simulink subsystem "Autonomous_sub"  (R2023b)
settings: Solver=VariableStepAuto  StartTime=0.0  StopTime=10.0  RelTol=1e-3
undefined symbols (not defined in the file): Auto_Deploy_Intake_Time, Auto_Deploy_Intake_Time2, Auto_Intake_Arm_Cycle_Delay_Time, Auto_Path_01, Auto_Path_02, Auto_Path_03, Auto_Path_04, Auto_Path_05, Auto_Path_06, Auto_Path_07, Auto_Path_08, Auto_Path_09, Auto_Path_10, Auto_Path_11, Auto_Path_12, Auto_Path_13, Auto_Path_Chooser, Auto_Shoot_Time, t_sample
libraries: simulink x11
settings Model: Creator=ander  LastModifiedBy=ander

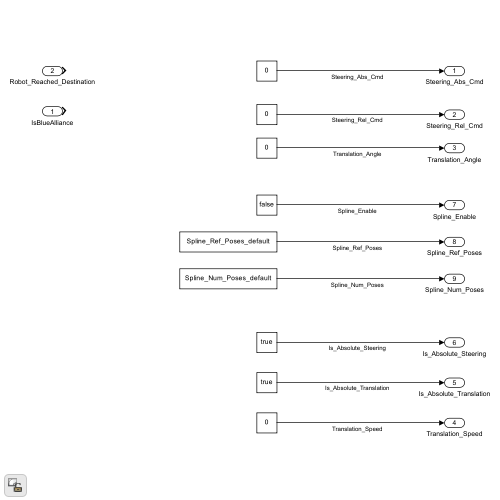
[thumbnail: Simulink's stored preview of the top-level diagram]
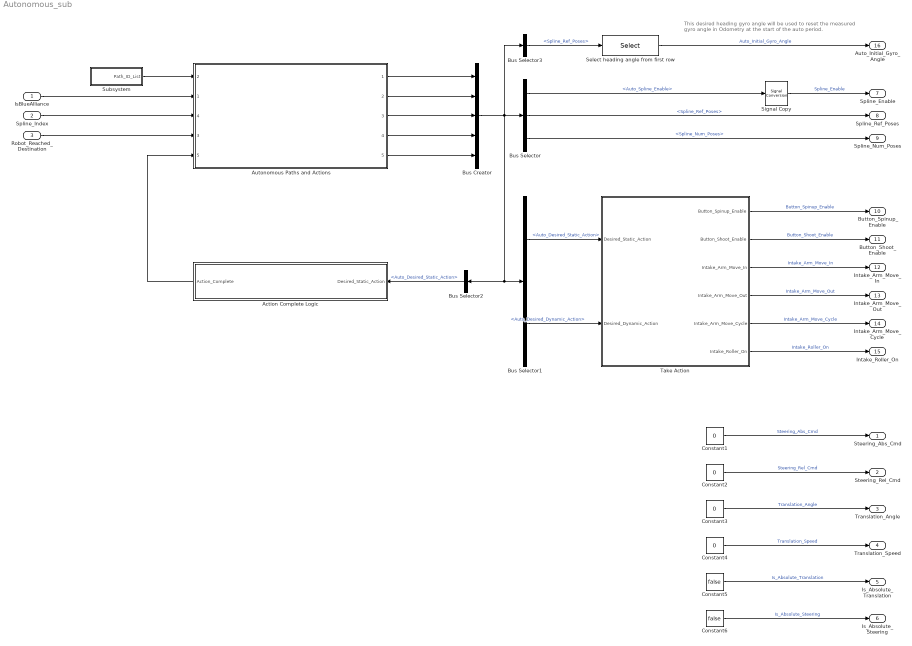
== system Autonomous_sub ==
  note: This desired heading gyro angle will be used to reset the measured gyro angle in Odometry at the start of the auto period.
  IsBlueAlliance : Inport
  Spline_Index : Inport  Port=2
  Robot_Reached_Destination : Inport  Port=3
  Action Complete Logic : Subsystem
  Autonomous Paths and Actions : Subsystem  ReferencedSubsystem=Autonomous_Paths_and_Actions_sub
      settings: PortSchema="{\"entries\":[{\"content\":{\"sides\":[{\"content\":{\"connectorIds\":[\"In2\",\"In1\",\"In4\",\"In3\",\"In5\"]},\"type\":\"ConnectorPlacement.EquallySpacedRectSide\",\"uuid\":\"294b2687-843c-4c6b-bb7a-4ddaa154855b\"},{\"content\":{\"connectorIds\":[\"Out1\",\"Out2\",\"Out3\",\"Out4\",\"Out5\"],\"side\":\"RIGHT\"},\"type\":\"ConnectorPlacement.EquallySpacedRectSide\",\"uuid\":\"d2e82f95-38dc-427a-93e1-a9041617c293\"},{\"content\":{\"side\":\"TOP\"},\"type\":\"ConnectorPlacement.EquallySpacedRectSide\",\"uuid\":\"31522bff-3666-4a04-81e4-ecf410bf1187\"}]},\"type\":\"ConnectorPlacement.EquallySpacedConnector\",\"uuid\":\"964fa79a-4b4c-4d0b-bc10-97a47e67b0ba\"}],\"packageUris\":[\"http://schema.mathworks.com/mf0/Connector/R2020b\"],\"version\":\"1.0\"}"
  Bus Creator : BusCreator  Inputs=5
  Bus Selector : BusSelector  OutputSignals=Auto_Spline_Enable,Spline_Ref_Poses,Spline_Num_Poses
  Bus Selector1 : BusSelector  OutputSignals=Auto_Desired_Static_Action,Auto_Desired_Dynamic_Action
  Bus Selector2 : BusSelector  OutputSignals=Auto_Desired_Static_Action
  Bus Selector3 : BusSelector  OutputSignals=Spline_Ref_Poses
  Constant{1..4} (4 alike) : Constant  Value=0
  Constant5 : Constant  Value=false
  Constant6 : Constant  Value=false
  Select heading angle from first row : Selector  NumberOfDimensions=2  InputPortWidth=3  IndexOptions=Index vector (dialog),Index vector (dialog)  Indices=[1],[4]  OutputSizes=1,1
  Signal Copy : SignalConversion  OverrideOpt=off
  Subsystem : Subsystem
  Take Action : Subsystem
  Steering_Abs_Cmd : Outport
  Steering_Rel_Cmd : Outport  Port=2
  Translation_Angle : Outport  Port=3
  Translation_Speed : Outport  Port=4
  Is_Absolute_Translation : Outport  Port=5
  Is_Absolute_Steering : Outport  Port=6
  Spline_Enable : Outport  Port=7
  Spline_Ref_Poses : Outport  Port=8
  Spline_Num_Poses : Outport  Port=9
  Button_Spinup_Enable : Outport  Port=10
  Button_Shoot_Enable : Outport  Port=11
  Intake_Arm_Move_In : Outport  Port=12
  Intake_Arm_Move_Out : Outport  Port=13
  Intake_Arm_Move_Cycle : Outport  Port=14
  Intake_Roller_On : Outport  Port=15
  Auto_Initial_Gyro_Angle : Outport  Port=16
  wires:
  Take Action/5(Intake_Arm_Move_Cycle) -> Intake_Arm_Move_Cycle/1  "Intake_Arm_Move_Cycle"
  Take Action/1(Button_Spinup_Enable) -> Button_Spinup_Enable/1  "Button_Spinup_Enable"
  Take Action/6(Intake_Roller_On) -> Intake_Roller_On/1  "Intake_Roller_On"
  Take Action/2(Button_Shoot_Enable) -> Button_Shoot_Enable/1  "Button_Shoot_Enable"
  Take Action/4(Intake_Arm_Move_Out) -> Intake_Arm_Move_Out/1  "Intake_Arm_Move_Out"
  Take Action/3(Intake_Arm_Move_In) -> Intake_Arm_Move_In/1  "Intake_Arm_Move_In"
  Bus Creator/1 -> Bus Selector/1, Bus Selector2/1, Bus Selector1/1, Bus Selector3/1
  Robot_Reached_Destination/1 -> Autonomous Paths and Actions/3
  Autonomous Paths and Actions/5 -> Bus Creator/5
  Autonomous Paths and Actions/4 -> Bus Creator/4
  Autonomous Paths and Actions/3 -> Bus Creator/3
  Autonomous Paths and Actions/1 -> Bus Creator/1
  Autonomous Paths and Actions/2 -> Bus Creator/2
  Constant5/1 -> Is_Absolute_Translation/1  "Is_Absolute_Translation"
  Bus Selector/1 -> Signal Copy/1  "<Auto_Spline_Enable>"
  Constant6/1 -> Is_Absolute_Steering/1  "Is_Absolute_Steering"
  Constant3/1 -> Translation_Angle/1  "Translation_Angle"
  Constant4/1 -> Translation_Speed/1  "Translation_Speed"
  Constant2/1 -> Steering_Rel_Cmd/1  "Steering_Rel_Cmd"
  Constant1/1 -> Steering_Abs_Cmd/1  "Steering_Abs_Cmd"
  Bus Selector/2 -> Spline_Ref_Poses/1  "<Spline_Ref_Poses>"
  Bus Selector/3 -> Spline_Num_Poses/1  "<Spline_Num_Poses>"
  Subsystem/1(Path_ID_List) -> Autonomous Paths and Actions/2
  Spline_Index/1 -> Autonomous Paths and Actions/4
  IsBlueAlliance/1 -> Autonomous Paths and Actions/1
  Bus Selector1/1 -> Take Action/1(Desired_Static_Action)  "<Auto_Desired_Static_Action>"
  Bus Selector1/2 -> Take Action/2(Desired_Dynamic_Action)  "<Auto_Desired_Dynamic_Action>"
  Bus Selector2/1 -> Action Complete Logic/1(Desired_Static_Action)  "<Auto_Desired_Static_Action>"
  Action Complete Logic/1(Action_Complete) -> Autonomous Paths and Actions/5
  Signal Copy/1 -> Spline_Enable/1  "Spline_Enable"
  Bus Selector3/1 -> Select heading angle from first row/1  "<Spline_Ref_Poses>"
  Select heading angle from first row/1 -> Auto_Initial_Gyro_Angle/1  "Auto_Initial_Gyro_Angle"

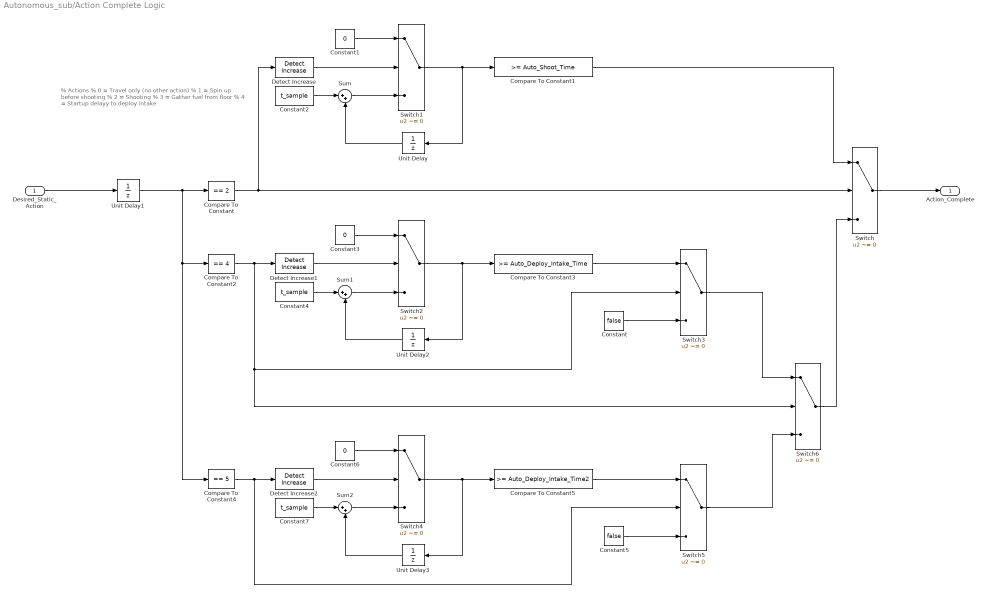
== system Autonomous_sub/Action Complete Logic ==
  note: % Actions
      | % 0 = Travel only (no other action)
      | % 1 = Spin up before shooting
      | % 2 = Shooting
      | % 3 = Gather fuel from floor
      | % 4 = Startup delayy to deploy intake
  Desired_Static_Action : Inport
  Compare To Constant : simulink/Logic and Bit Operations/Compare To Constant  relop===  const=2  OutDataTypeStr=boolean
  Compare To Constant1 : simulink/Logic and Bit Operations/Compare To Constant  relop=>=  const=Auto_Shoot_Time  OutDataTypeStr=boolean
  Compare To Constant2 : simulink/Logic and Bit Operations/Compare To Constant  relop===  const=4  OutDataTypeStr=boolean
  Compare To Constant3 : simulink/Logic and Bit Operations/Compare To Constant  relop=>=  const=Auto_Deploy_Intake_Time  OutDataTypeStr=boolean
  Compare To Constant4 : simulink/Logic and Bit Operations/Compare To Constant  relop===  const=5  OutDataTypeStr=boolean
  Compare To Constant5 : simulink/Logic and Bit Operations/Compare To Constant  relop=>=  const=Auto_Deploy_Intake_Time2  OutDataTypeStr=boolean
  Constant : Constant  Value=false
  Constant1 : Constant  Value=0
  Constant2 : Constant  Value=t_sample
  Constant3 : Constant  Value=0
  Constant4 : Constant  Value=t_sample
  Constant5 : Constant  Value=false
  Constant6 : Constant  Value=0
  Constant7 : Constant  Value=t_sample
  Detect Increase : simulink/Logic and Bit Operations/Detect Increase  vinit=0.0  OutDataTypeStr=boolean
  Detect Increase1 : simulink/Logic and Bit Operations/Detect Increase  vinit=0.0  OutDataTypeStr=boolean
  Detect Increase2 : simulink/Logic and Bit Operations/Detect Increase  vinit=0.0  OutDataTypeStr=boolean
  Sum : Sum  Inputs=|++
  Sum1 : Sum  Inputs=|++
  Sum2 : Sum  Inputs=|++
  Switch{,1..6} (7 alike) : Switch  Criteria=u2 ~= 0  SaturateOnIntegerOverflow=off  InputSameDT=off
  Unit Delay{,1..3} (4 alike) : UnitDelay  SampleTime=-1  HasFrameUpgradeWarning=on
  Action_Complete : Outport
  wires:
  Switch6/1 -> Switch/3
  Switch5/1 -> Switch6/3
  Switch3/1 -> Switch6/1
  Constant7/1 -> Sum2/1
  Unit Delay3/1 -> Sum2/2
  Sum2/1 -> Switch4/3
  Detect Increase2/1 -> Switch4/2
  Switch4/1 -> Compare To Constant5/1, Unit Delay3/1
  Constant6/1 -> Switch4/1
  Compare To Constant4/1 -> Switch5/2, Detect Increase2/1
  Compare To Constant5/1 -> Switch5/1
  Constant5/1 -> Switch5/3
  Constant/1 -> Switch3/3
  Compare To Constant3/1 -> Switch3/1
  Compare To Constant2/1 -> Detect Increase1/1, Switch3/2, Switch6/2
  Constant3/1 -> Switch2/1
  Switch2/1 -> Unit Delay2/1, Compare To Constant3/1
  Detect Increase1/1 -> Switch2/2
  Sum1/1 -> Switch2/3
  Unit Delay2/1 -> Sum1/2
  Constant4/1 -> Sum1/1
  Unit Delay1/1 -> Compare To Constant/1, Compare To Constant2/1, Compare To Constant4/1
  Compare To Constant1/1 -> Switch/1
  Unit Delay/1 -> Sum/2
  Switch1/1 -> Unit Delay/1, Compare To Constant1/1
  Constant2/1 -> Sum/1
  Sum/1 -> Switch1/3
  Constant1/1 -> Switch1/1
  Detect Increase/1 -> Switch1/2
  Switch/1 -> Action_Complete/1
  Compare To Constant/1 -> Switch/2, Detect Increase/1
  Desired_Static_Action/1 -> Unit Delay1/1

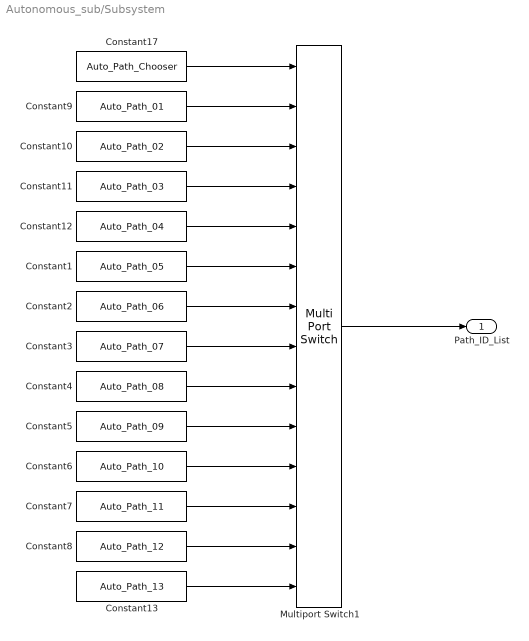
== system Autonomous_sub/Subsystem ==
  Constant1 : Constant  Value=Auto_Path_05
  Constant10 : Constant  Value=Auto_Path_02
  Constant11 : Constant  Value=Auto_Path_03
  Constant12 : Constant  Value=Auto_Path_04
  Constant13 : Constant  Value=Auto_Path_13
  Constant17 : Constant  Value=Auto_Path_Chooser
  Constant2 : Constant  Value=Auto_Path_06
  Constant3 : Constant  Value=Auto_Path_07
  Constant4 : Constant  Value=Auto_Path_08
  Constant5 : Constant  Value=Auto_Path_09
  Constant6 : Constant  Value=Auto_Path_10
  Constant7 : Constant  Value=Auto_Path_11
  Constant8 : Constant  Value=Auto_Path_12
  Constant9 : Constant  Value=Auto_Path_01
  Multiport Switch1 : MultiPortSwitch  Inputs=13  SaturateOnIntegerOverflow=off  InputSameDT=off
  Path_ID_List : Outport
  wires:
  Constant13/1 -> Multiport Switch1/14
  Constant8/1 -> Multiport Switch1/13
  Constant7/1 -> Multiport Switch1/12
  Constant6/1 -> Multiport Switch1/11
  Constant5/1 -> Multiport Switch1/10
  Constant4/1 -> Multiport Switch1/9
  Constant3/1 -> Multiport Switch1/8
  Constant2/1 -> Multiport Switch1/7
  Constant1/1 -> Multiport Switch1/6
  Multiport Switch1/1 -> Path_ID_List/1
  Constant9/1 -> Multiport Switch1/2
  Constant17/1 -> Multiport Switch1/1
  Constant11/1 -> Multiport Switch1/4
  Constant12/1 -> Multiport Switch1/5
  Constant10/1 -> Multiport Switch1/3

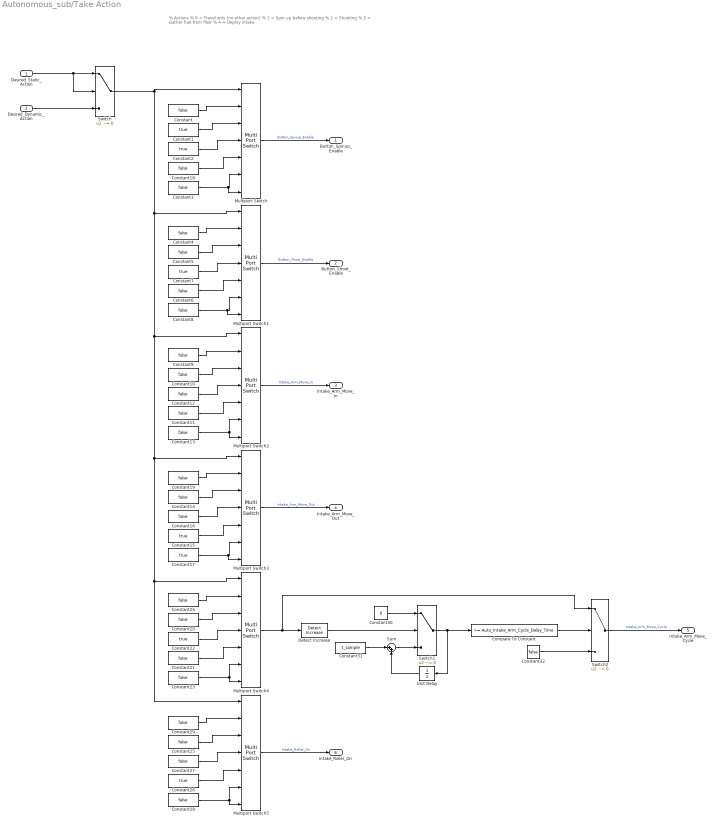
== system Autonomous_sub/Take Action ==
  note: % Actions
      | % 0 = Travel only (no other action)
      | % 1 = Spin up before shooting
      | % 2 = Shooting
      | % 3 = Gather fuel from floor
      | % 4 = Deploy intake
  Desired_Static_Action : Inport
  Desired_Dynamic_Action : Inport  Port=2
  Compare To Constant : simulink/Logic and Bit Operations/Compare To Constant  relop=>=  const=Auto_Intake_Arm_Cycle_Delay_Time  OutDataTypeStr=boolean
  Constant{,3..6,8..14,16,18..21,23..25,27..29,32} (24 alike) : Constant  Value=false
  Constant{1..2,7,15,17,22,26} (7 alike) : Constant  Value=true
  Constant30 : Constant  Value=0
  Constant31 : Constant  Value=t_sample
  Detect Increase : simulink/Logic and Bit Operations/Detect Increase  vinit=0.0  OutDataTypeStr=boolean
  Multiport Switch{,1..5} (6 alike) : MultiPortSwitch  DataPortOrder=Zero-based contiguous  Inputs=6  zeroidx=on  SaturateOnIntegerOverflow=off  InputSameDT=off
  Sum : Sum  Inputs=|++
  Switch : Switch  Criteria=u2 ~= 0  SaturateOnIntegerOverflow=off  InputSameDT=off
  Switch1 : Switch  Criteria=u2 ~= 0  SaturateOnIntegerOverflow=off  InputSameDT=off
  Switch2 : Switch  Criteria=u2 ~= 0  SaturateOnIntegerOverflow=off  InputSameDT=off
  Unit Delay : UnitDelay  SampleTime=-1  HasFrameUpgradeWarning=on
  Button_Spinup_Enable : Outport
  Button_Shoot_Enable : Outport  Port=2
  Intake_Arm_Move_In : Outport  Port=3
  Intake_Arm_Move_Out : Outport  Port=4
  Intake_Arm_Move_Cycle : Outport  Port=5
  Intake_Roller_On : Outport  Port=6
  wires:
  Multiport Switch4/1 -> Detect Increase/1, Switch2/1
  Switch2/1 -> Intake_Arm_Move_Cycle/1  "Intake_Arm_Move_Cycle"
  Constant32/1 -> Switch2/3
  Compare To Constant/1 -> Switch2/2
  Unit Delay/1 -> Sum/2
  Switch1/1 -> Unit Delay/1, Compare To Constant/1
  Constant31/1 -> Sum/1
  Sum/1 -> Switch1/3
  Constant30/1 -> Switch1/1
  Detect Increase/1 -> Switch1/2
  Multiport Switch5/1 -> Intake_Roller_On/1  "Intake_Roller_On"
  Multiport Switch3/1 -> Intake_Arm_Move_Out/1  "Intake_Arm_Move_Out"
  Multiport Switch2/1 -> Intake_Arm_Move_In/1  "Intake_Arm_Move_In"
  Multiport Switch1/1 -> Button_Shoot_Enable/1  "Button_Shoot_Enable"
  Constant26/1 -> Multiport Switch5/5
  Constant27/1 -> Multiport Switch5/4
  Constant29/1 -> Multiport Switch5/2
  Constant28/1 -> Multiport Switch5/6, Multiport Switch5/7
  Constant25/1 -> Multiport Switch5/3
  Constant20/1 -> Multiport Switch4/3
  Constant23/1 -> Multiport Switch4/6, Multiport Switch4/7
  Constant24/1 -> Multiport Switch4/2
  Constant22/1 -> Multiport Switch4/4
  Constant21/1 -> Multiport Switch4/5
  Constant15/1 -> Multiport Switch3/5
  Constant16/1 -> Multiport Switch3/4
  Constant19/1 -> Multiport Switch3/2
  Constant17/1 -> Multiport Switch3/6, Multiport Switch3/7
  Constant14/1 -> Multiport Switch3/3
  Constant10/1 -> Multiport Switch2/3
  Constant13/1 -> Multiport Switch2/7, Multiport Switch2/6
  Constant9/1 -> Multiport Switch2/2
  Constant12/1 -> Multiport Switch2/4
  Constant11/1 -> Multiport Switch2/5
  Constant4/1 -> Multiport Switch1/2
  Constant5/1 -> Multiport Switch1/3
  Constant7/1 -> Multiport Switch1/4
  Constant6/1 -> Multiport Switch1/5
  Constant8/1 -> Multiport Switch1/6, Multiport Switch1/7
  Constant3/1 -> Multiport Switch/6, Multiport Switch/7
  Constant18/1 -> Multiport Switch/5
  Constant2/1 -> Multiport Switch/4
  Constant1/1 -> Multiport Switch/3
  Constant/1 -> Multiport Switch/2
  Switch/1 -> Multiport Switch/1, Multiport Switch2/1, Multiport Switch3/1, Multiport Switch4/1, Multiport Switch5/1, Multiport Switch1/1
  Desired_Dynamic_Action/1 -> Switch/3
  Desired_Static_Action/1 -> Switch/1, Switch/2
  Multiport Switch/1 -> Button_Spinup_Enable/1  "Button_Spinup_Enable"
